simulink model "sfGetStartedFlowchart"  (R2025b)
settings: Solver=VariableStepAuto  StartTime=0.0  StopTime=10.0  RelTol=1e-3
settings Model: Creator=The MathWorks, Inc.  LastModifiedBy=The MathWorks, Inc.

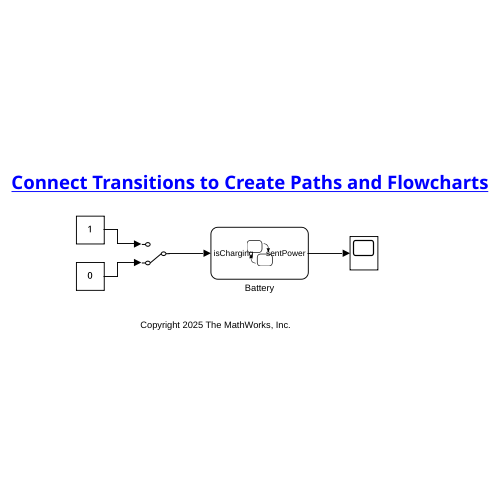
[thumbnail: Simulink's stored preview of the top-level diagram]
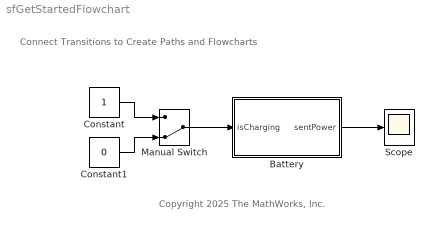
== system sfGetStartedFlowchart ==
  note: Copyright 2025 The MathWorks, Inc.
  note: Connect Transitions to Create Paths and Flowcharts
  Battery : Stateflow chart  TreatAsAtomicUnit=on
  Constant : Constant
  Constant1 : Constant  Value=0
  Manual Switch : ManualSwitch  CurrentSetting=0
  Scope : Scope
      settings: ActiveDisplayYMinimum=-0.43749999999999989  ActiveDisplayYMaximum=3.9375
  wires:
  Manual Switch/1 -> Battery/1(isCharging)
  Constant/1 -> Manual Switch/1
  Constant1/1 -> Manual Switch/2
  Battery/1(sentPower) -> Scope/1

== stateflow chart sfGetStartedFlowchart/Battery ==
  state Charge
    entry:
    sentPower=0;
    state FastCharge
      during:
      charge=charge+4;
    state SlowCharge
      during:
      charge=charge+1;
    state Full
    (default) -> FastCharge
    FastCharge -> SlowCharge : [charge>80]
    SlowCharge -> Full : [charge==100]
  state Discharge
    entry:
    sentPower=3.5;
    state Powered
      during:
      charge=charge-3;
    state Empty
      entry:
      sentPower=0;
    (default) -> Powered
    Powered -> Empty : [charge<=3]
  (default) -> Charge
  Charge -> Discharge : [~isCharging]
  Discharge -> Charge : [isCharging]
  data: isCharging input; sentPower output; charge local =50
